simulink model "fuelcell"  (R2024a)
settings: Solver=VariableStepAuto  StartTime=0.0  StopTime=0.025  RelTol=1e-3
libraries: spsCurrentMeasurementLib x1, spsFuelCellStackLib x1, simulink x1, spsVariableResistorLib x1, spsVoltageMeasurementLib x1, spspowerguiLib x1
settings Model: Creator=LOUZAZNI  LastModifiedBy=Aswin
settings SolverCC: AlgebraicLoopSolver=TrustRegion
settings DebuggingCC: UnconnectedInputMsg=warning  UnconnectedOutputMsg=warning  UnconnectedLineMsg=warning
settings ModelReferenceCC: EnableRefExpFcnMdlSchedulingChecks=on
settings SFSimCC: CustomCodeUndefinedFunction=UseInterfaceOnly
settings RTWCC: GPUComputeCapability=3.5

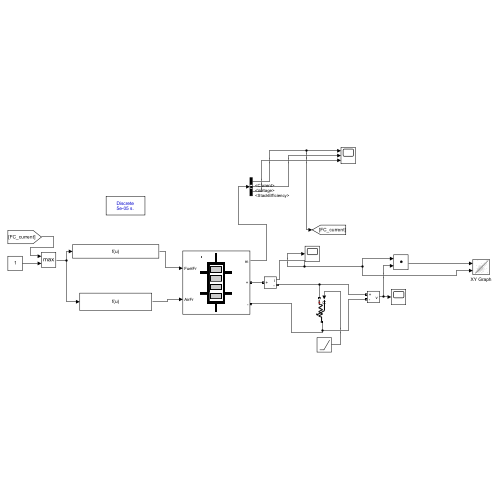
[thumbnail: Simulink's stored preview of the top-level diagram]
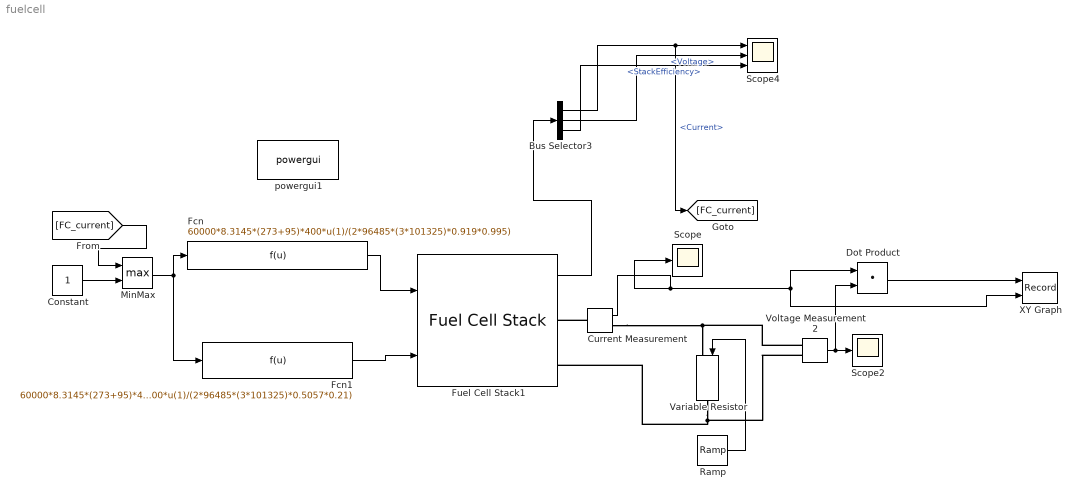
== system fuelcell ==
  Bus Selector3 : BusSelector  OutputSignals=Current,Voltage,StackEfficiency
  Constant : Constant
  Current Measurement : spsCurrentMeasurementLib/Current Measurement  PhasorSimulation=off  OutputType=Complex  PSBequivalent=0
  Dot Product : DotProduct  OutDataTypeStr=Inherit: Inherit via internal rule
  Fcn : Fcn  Expr=60000*8.3145*(273+95)*400*u(1)/(2*96485*(3*101325)*0.919*0.995)
  Fcn1 : Fcn  Expr=60000*8.3145*(273+95)*400*u(1)/(2*96485*(3*101325)*0.5057*0.21)
  Fuel Cell Stack1 : spsFuelCellStackLib/Fuel Cell Stack  PresetModel=PEMFC - 6 kW - 45 Vdc  FcType=Proton Exchange Membrane (PEM)  Detailed=Detailed  Eoc=[65,63]  NomVI=[133.3,45]  EndVI=[225,37]  Nc=65  n=55  TOp=65  AirFr=300  SuppPress=[1.5,1]  Comp=[99.95,21,1]  SignX=off  SignY=off  FlowRateH2=on  FlowRateAir=on  SystemTemp=off  SystemPH2=off  SystemPAir=off  FCDyn=off  FC_tau=0  Peak_O2=80  V_Under=10
      settings: LibrarySourceBlock=electricdrivelib/Extra Sources/Fuel Cell Stack
  MinMax : MinMax  Function=max  Inputs=2
  Ramp : simulink/Sources/Ramp  slope=0.25  start=0  InitialOutput=0
  Scope : Scope
  Scope2 : Scope
  Scope4 : Scope  NumInputPorts=3
  Variable Resistor : spsVariableResistorLib/Variable Resistor  Rabsmin=1e-3
      settings: LibrarySourceBlock=sps_lib/Passives/Variable Resistor
  Voltage Measurement2 : spsVoltageMeasurementLib/Voltage Measurement  PhasorSimulation=off  OutputType=Complex  PSBequivalent=0
  XY Graph : Record  FileSettingsInternal="{\"entries\":[{\"content\":{\"excelSettings\":{\"content\":{},\"type\":\"Streamout.ExcelSettings\"}},\"type\":\"Streamout.FileSettingStorage\",\"uuid\":\"\"}],\"packageUris\":[\"http:\\/\\/schema.mathworks.com\\/mf0\\/streamout_blocks\\/R2020a\"],\"version\":\"1.0\"}"  Layout=[1 1]  SignalsInternal="{\"entries\":[{\"content\":{\"signals\":[{\"content\":{\"blockPath\":[],\"dimensions\":[1],\"domain\":\"\",\"lineColor\":\"#a2142f\",\"plots\":[ 1 ],\"port\":1,\"signalID\":1,\"signalName\":\"Dot Product\"},\"type\":\"RecordBlkView.Signal\",\"uuid\":\"\"},{\"content\":{\"blockPath\":[],\"dimensions\":[1],\"domain\":\"\",\"lineColor\":\"#139fff\",\"plots\":[ 1 ],\"port\":2,\"signalID\":2,\"signalName\":\"Current Measurement\"},\"type\":\"RecordBlkView.Signal\",\"uuid\":\"\"}]},\"type\":\"RecordBlkView.InputSignals\",\"uuid\":\"\"}],\"packageUris\":[\"http:\\/\\/schema.mathworks.com\\/mf0\\/streamout_blocks\\/R2020a\"],\"version\":\"1.0\"}"  VisualizationBindings="{\"xyplotplugin\":{\"info\":[{\"series\":[{\"bindingParametersList\":[{\"parameter\":\"X-Axis\",\"signalID\":2,\"signalName\":\"Current Measurement\"},{\"parameter\":\"Y-Axis\",\"signalID\":1,\"signalName\":\"Dot Product\"}],\"seriesID\":0}],\"subplotID\":1}]}}"  CompatibilityTag=XY
  powergui1 : spspowerguiLib/powergui  Priority=1  SimulationMode=Discrete  SampleTime=50e-6  frequency=60  Iterations=50  frequencyindice=0  Pbase=100e6  ErrMax=1e-4  UnitsV=kV  UnitsW=MW  buscounter=0  FunctionMessages=off  echomessages=off  EnableUseOfTLC=off  CurrentSourceSwitches=off  DisableSnubberDevices=off  DisableRonSwitches=off  DisableVfSwitches=off  DisplayEquations=off  AutomaticDiscreteSolvers=off  SolverType=Tustin/Backward Euler (TBE)  Interpol=off  ExternalGateDelay=off  methode=off  Ts=100  x0status=blocks  SPID=on  SwTol=0  HookPort=off  NonlinearTolerance=1e-4  nMaxIteration=100  ContinueOnMaxIteration=off  RestoreLinks=warning  ResistiveCurrentMeasurement=off  Frange=[0:2:500]  Ylog=off  Xlog=on  ShowGrid=off  save=off  variable=ZData  structure=0  ZoomFFT=off  StartTime=0.0  cycles=1  DisplayStyle=1  fundamental=60  FreqAxis=off  MaxFrequency=1000  frequencyindicesteady=1  RmsSteady=1  display=off
  wires:
  Fuel Cell Stack1/1 -> Bus Selector3/1
  MinMax/1 -> Fcn1/1, Fcn/1
  Fcn/1 -> Fuel Cell Stack1/1
  Fcn1/1 -> Fuel Cell Stack1/2
  [FC_current] -> MinMax/1
  Constant/1 -> MinMax/2
  Bus Selector3/1 -> [FC_current], Scope4/1  "<Current>"
  Bus Selector3/2 -> Scope4/2  "<Voltage>"
  Bus Selector3/3 -> Scope4/3  "<StackEfficiency>"
  Voltage Measurement2/1 -> Dot Product/2, Scope2/1
  Ramp/1 -> Variable Resistor/1
  Current Measurement/1 -> XY Graph/2, Dot Product/1, Scope/1
  Dot Product/1 -> XY Graph/1
  connections:
  Voltage Measurement2/LConn1 -- Current Measurement/RConn1 -- Variable Resistor/LConn1
  Voltage Measurement2/LConn2 -- Variable Resistor/RConn1 -- Fuel Cell Stack1/RConn2
  Current Measurement/LConn1 -- Fuel Cell Stack1/RConn1
